simulink model "Fixed_Base_Simulation"  (R2026b)
settings: Solver=ode23t  StopTime=25  MaxStep=0.01
InitFcn:
  | GeneratePointGrid
model workspace (MAT data in the model file):
  MW_MaxNumBodies = 100
  MW_MaxNumCollisions = 5
  MW_MaxNumVertices = 10000
undefined symbols (not defined in the file): t_s
libraries: simulink x1
settings Model: Creator=Janelyn Anderson  LastModifiedBy=Janelyn Anderson
settings OptimizationCC: DefaultParameterBehavior=Inlined  DifferentSizesBufferReuse=on  EfficientFloat2IntCast=on  EfficientTunableParamExpr=on  EnhancedBackFolding=on  InlineInvariantSignals=on  LifeSpan=inf  OptimizationCustomize=off  OptimizeBlockOrder=speed  PassReuseOutputArgsAs=Individual arguments  RemoveInternalMemoryZeroInit=on  RemoveRootLevelIOMemoryZeroInit=on  UseDivisionForNetSlopeComputation=UseDivisionForReciprocalsOfIntegersOnly
settings DebuggingCC: AssertControl=DisableAll  ParameterTunabilityLossMsg=error  SignalInfNanChecking=warning
settings HardwareCC: ProdHWDeviceType=ARM Compatible->ARM Cortex-M  ProdLargestAtomicFloat=Double  ProdLargestAtomicInteger=Long  ProdShiftRightIntArith=off
settings SFSimCC: EnableRuntimeRecursion=off  MATLABDynamicMemAlloc=off
settings RTWCC: DataTypeReplacement=CDataTypesFixedWidth  Description=Teensy ERT Target  SystemTargetFile=teensy_ert.tlc  TemplateMakefile=teensy_ert.tmf
settings CodeAppCC: ForceParamTrailComments=on  IgnoreCustomStorageClasses=off  IgnoreTestpoints=on  InsertBlockDesc=on  MATLABFcnDesc=on  OperatorAnnotations=on  SFDataObjDesc=on  SimulinkDataObjDesc=on
settings STFCustomTargetCC: CPPClassGenCompliant=on  CastingMode=Standards  CombineOutputUpdateFcns=on  CombineSignalStateStructs=on  ERTCustomFileBanners=on  GRTInterface=off  GenerateSampleERTMain=on  GenerateSharedConstants=off  MATLABClassNameForMDSCustomization=Simulink.SoftwareTarget.ERTCustomization  ParenthesesLevel=Standards  RemoveResetFunc=on  SupportContinuousTime=off  SupportNonFinite=off  SupportNonInlinedSFcns=off  SuppressErrorStatus=on  SystemTargetFile=teensy_ert.tlc  TargetLibSuffix=.a  UtilityFuncGeneration=Shared location
settings ERTTargetCC: CastingMode=Standards  CombineSignalStateStructs=on  CompOptLevelCompliant=off  ConcurrentExecutionCompliant=off  ERTCustomFileTemplate=teensy_ert_file_process.tlc  EnableSignedLeftShifts=off  EnableSignedRightShifts=off  ExtModeMexArgs=0 1 4000000  ExtModeMexFile=ext_serial_win32_comm  GenerateSampleERTMain=on  GenerateSharedConstants=off  MaxIdInt16=INT16_MAX  MaxIdInt32=INT32_MAX  MaxIdInt64=INT64_MAX  MaxIdInt8=INT8_MAX  MaxIdUint16=UINT16_MAX  MaxIdUint32=UINT32_MAX  MaxIdUint64=UINT64_MAX  MaxIdUint8=UINT8_MAX  MinIdInt16=INT16_MIN  MinIdInt32=INT32_MIN  MinIdInt64=INT64_MIN  MinIdInt8=INT8_MIN  ModelStepFunctionPrototypeControlCompliant=off  ParMdlRefBuildCompliant=off  ParenthesesLevel=Standards  SupportNonFinite=off  SuppressErrorStatus=on  UtilityFuncGeneration=Shared location
settings SimscapeCC: SimscapeLogType=all  SimscapeNominalValues="[{\"value\":\"1\",\"unit\":\"A\"},{\"value\":\"1\",\"unit\":\"bar\"},{\"value\":\"1\",\"unit\":\"cm^2\"},{\"value\":\"1\",\"unit\":\"cm^3/s\"},{\"value\":\"1\",\"unit\":\"kJ/kg\"},{\"value\":\"1\",\"unit\":\"kW\"},{\"value\":\"1\",\"unit\":\"l\"},{\"value\":\"1\",\"unit\":\"N\"},{\"value\":\"1\",\"unit\":\"N*m\"},{\"value\":\"1\",\"unit\":\"V\"},{\"value\":\"0.001\",\"unit\":\"Wb\"}]"  SimscapeUseEnergyAccounting=off
settings ExplorerConfigSet: InternalSimMechanicsExplorerSettings=|
  | <ExplorerConfiguration>
  | 
  |   <canonicalview>default</canonicalview>
  | 
  |   <TilePanel>
  |     <TileInfo>
  |       <Tiles Columns="1" Count="1" Height="706" Rows="1" Width="1046">
  |         <Row Weight="1"/>
  |         <Column Weight="1"/>
  |         <Tile Height="1" Width="1" X="0" Y="0"/>
  |       </Tiles>
  |     </TileInfo>
  |     <SceneInfo>
  |       <SceneViewer>
  |         <IsThisViewStd>
  |           <IsStandardView>off</IsStandardView>
  |           <StandardViewName>Front</StandardViewName>
  |         </IsThisViewStd>
  |         <BGColor>
  |           <R>1</R>
  |           <G>1</G>
  |           <B>1</B>
  |           <A>1</A>
  |         </BGColor>
  |         <Camera>
  |           <DoPerspective>off</DoPerspective>
  |           <Position>
  |             <X>-2.5213345787478829</X>
  |             <Y>-2.7245462411520407</Y>
  |             <Z>2.904483486867131</Z>
  |           </Position>
  |           <Center>
  |             <X>0.10443685676261794</X>
  |             <Y>-0.098774805641539842</Y>
  |             <Z>0.27871205135663013</Z>
  |           </Center>
  |           <Up>
  |             <X>0.40824829046386307</X>
  |             <Y>0.40824829046386307</Y>
  |             <Z>0.81649658092772615</Z>
  |           </Up>
  |           <XLim>0.4230568512943666</XLim>
  |           <YLim>0.4230568512943666</YLim>
  |           <ViewLimDist>0.01</ViewLimDist>
  |         </Camera>
  |       </SceneViewer>
  |     </SceneInfo>
  |   </TilePanel>
  | 
  |   <MechEditorPanel>
  |     <GfxPanelCameraMap/>
  |     <Cameras/>
  |     <VideoCreator>
  |       <IncludeTiles>All</IncludeTiles>
  |       <IncludeTime>on</IncludeTime>
  |       <IncludeWorldFrame>off</IncludeWorldFrame>
  |       <PlaybackSpeedRatio>1</PlaybackSpeedRatio>
  |       <FrameRate>30</FrameRate>
  |       <FrameSize>[1280, 720]</FrameSize>
  |       <VideoFormat>MPEG4</VideoFormat>
  |     </VideoCreator>
  |   </MechEditorPanel>
  | 
  |   <PlaybackSettings>
  |     <PlaybackSpeedFactor>1</PlaybackSpeedFactor>
  |   </PlaybackSettings>
  | 
  | </ExplorerConfiguration>

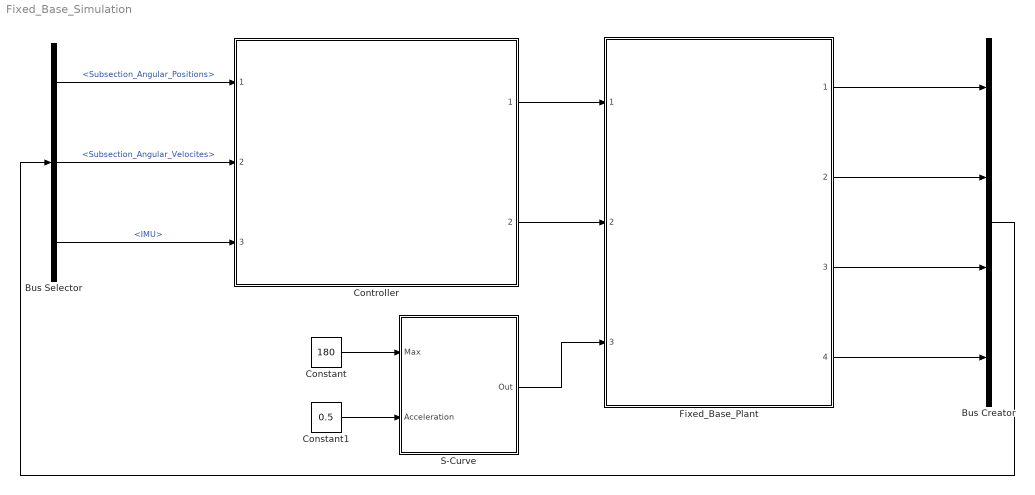
== system Fixed_Base_Simulation ==
  Bus Creator : BusCreator  Inputs=4
  Bus Selector : BusSelector  OutputSignals=Subsection_Angular_Positions,Subsection_Angular_Velocites,IMU
  Constant : Constant  Value=180
  Constant1 : Constant  Value=0.5
  Controller : Subsystem  ReferencedSubsystem=Top_Level_Controller
  Fixed_Base_Plant : Subsystem  ReferencedSubsystem=Fixed_Base_Plant
  S-Curve : Subsystem
  wires:
  Controller/1 -> Fixed_Base_Plant/1
  Fixed_Base_Plant/4 -> Bus Creator/4
  Fixed_Base_Plant/3 -> Bus Creator/3
  Fixed_Base_Plant/2 -> Bus Creator/2
  Fixed_Base_Plant/1 -> Bus Creator/1
  Bus Selector/2 -> Controller/2  "<Subsection_Angular_Velocites>"
  Bus Selector/1 -> Controller/1  "<Subsection_Angular_Positions>"
  Bus Creator/1 -> Bus Selector/1
  Controller/2 -> Fixed_Base_Plant/2
  Constant/1 -> S-Curve/1(Max)
  Constant1/1 -> S-Curve/2(Acceleration)
  S-Curve/1(Out) -> Fixed_Base_Plant/3
  Bus Selector/3 -> Controller/3  "<IMU>"

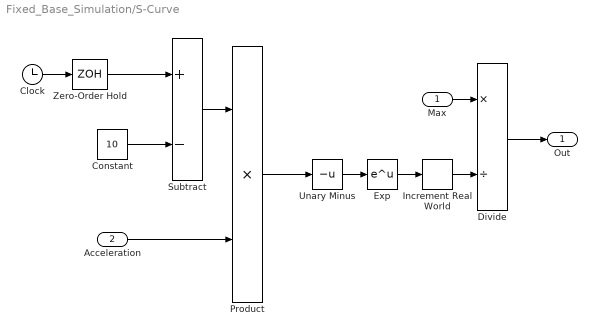
== system Fixed_Base_Simulation/S-Curve ==
  Max : Inport
  Acceleration : Inport  Port=2
  Clock : Clock
  Constant : Constant  Value=10
  Divide : Product  Inputs=*/
  Exp : Math
  Increment Real World : simulink/Additional Math & Discrete/Additional Math: Increment - Decrement/Increment Real World
  Product : Product
  Subtract : Sum  Inputs=+-
  Unary Minus : UnaryMinus
  Zero-Order Hold : ZeroOrderHold  SampleTime=t_s
  Out : Outport
  wires:
  Clock/1 -> Zero-Order Hold/1
  Constant/1 -> Subtract/2
  Subtract/1 -> Product/1
  Acceleration/1 -> Product/2
  Product/1 -> Unary Minus/1
  Unary Minus/1 -> Exp/1
  Exp/1 -> Increment Real World/1
  Increment Real World/1 -> Divide/2
  Max/1 -> Divide/1
  Divide/1 -> Out/1
  Zero-Order Hold/1 -> Subtract/1
